simulink model "solar_tracker"  (R2026b)
settings: Solver=ode4  StopTime=cfg.simulation.durationHours * 3600  FixedStep=cfg.simulation.energySampleTime
model workspace (MAT data in the model file):
  targetAzimuthInput = timeseries
  targetAzimuthInput.Name = 'unnamed'
  targetAzimuthInput.DataInfo = tsdata.datametadata
  targetAzimuthInput.DataInfo.Interpolation = tsdata.interpolation
  targetAzimuthInput.DataInfo.Interpolation.Fhandle : function handle (value not decoded)
  targetAzimuthInput.DataInfo.Interpolation.Name = 'linear'
  targetAzimuthInput.TimeInfo = tsdata.timemetadata
  targetAzimuthInput.TimeInfo.Length = 2
  targetAzimuthInput.TimeInfo.DuplicateTimes = 0
  targetAzimuthInput.TimeInfo.Time_ = [0; 86400]
  targetAzimuthInput.TimeInfo.Initialized = 1
  targetAzimuthInput.QualityInfo = tsdata.qualmetadata
  targetAzimuthInput.Data_ = [0; 0]
  targetTiltInput = timeseries
  targetTiltInput.Name = 'unnamed'
  targetTiltInput.DataInfo = tsdata.datametadata
  targetTiltInput.DataInfo.Interpolation = tsdata.interpolation
  targetTiltInput.DataInfo.Interpolation.Fhandle : function handle (value not decoded)
  targetTiltInput.DataInfo.Interpolation.Name = 'linear'
  targetTiltInput.TimeInfo = tsdata.timemetadata
  targetTiltInput.TimeInfo.Length = 2
  targetTiltInput.TimeInfo.DuplicateTimes = 0
  targetTiltInput.TimeInfo.Time_ = [0; 86400]
  targetTiltInput.TimeInfo.Initialized = 1
  targetTiltInput.QualityInfo = tsdata.qualmetadata
  targetTiltInput.Data_ = [0; 0]
values from neighbouring files (symbols this model uses):
  cfg = project_config()    [validate_tracker_plant.m]    (also in verify_axis_plant.m)
settings Model: Creator=Jhons Janner Samuel  LastModifiedBy=Jhons Janner Samuel

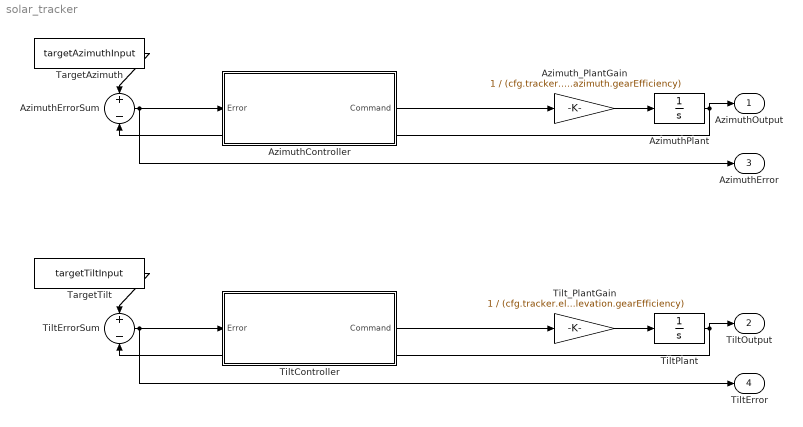
== system solar_tracker ==
  AzimuthController : Subsystem
  AzimuthErrorSum : Sum  Inputs=+-
  AzimuthPlant : Integrator
  Azimuth_PlantGain : Gain  Gain=1 / (cfg.tracker.azimuth.gearRatio * cfg.tracker.azimuth.gearEfficiency)
  TargetAzimuth : FromWorkspace  VariableName=targetAzimuthInput
  TargetTilt : FromWorkspace  VariableName=targetTiltInput
  TiltController : Subsystem
  TiltErrorSum : Sum  Inputs=+-
  TiltPlant : Integrator
  Tilt_PlantGain : Gain  Gain=1 / (cfg.tracker.elevation.gearRatio * cfg.tracker.elevation.gearEfficiency)
  AzimuthOutput : Outport
  TiltOutput : Outport  Port=2
  AzimuthError : Outport  Port=3
  TiltError : Outport  Port=4
  wires:
  TargetAzimuth/1 -> AzimuthErrorSum/1
  TargetTilt/1 -> TiltErrorSum/1
  AzimuthErrorSum/1 -> AzimuthController/1(Error), AzimuthError/1
  AzimuthController/1(Command) -> Azimuth_PlantGain/1
  Azimuth_PlantGain/1 -> AzimuthPlant/1
  AzimuthPlant/1 -> AzimuthOutput/1, AzimuthErrorSum/2
  TiltErrorSum/1 -> TiltController/1(Error), TiltError/1
  TiltController/1(Command) -> Tilt_PlantGain/1
  Tilt_PlantGain/1 -> TiltPlant/1
  TiltPlant/1 -> TiltOutput/1, TiltErrorSum/2

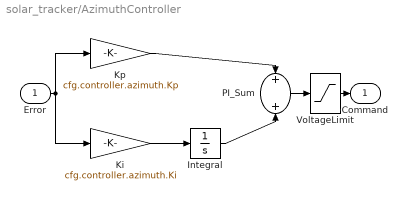
== system solar_tracker/AzimuthController ==
  Error : Inport
  Integral : Integrator
  Ki : Gain  Gain=cfg.controller.azimuth.Ki
  Kp : Gain  Gain=cfg.controller.azimuth.Kp
  PI_Sum : Sum
  VoltageLimit : Saturate  UpperLimit=cfg.controller.azimuth.outputMax  LowerLimit=cfg.controller.azimuth.outputMin
  Command : Outport
  wires:
  Error/1 -> Kp/1, Ki/1
  Ki/1 -> Integral/1
  Kp/1 -> PI_Sum/1
  Integral/1 -> PI_Sum/2
  PI_Sum/1 -> VoltageLimit/1
  VoltageLimit/1 -> Command/1

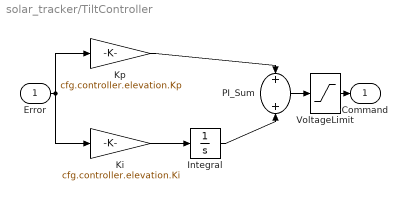
== system solar_tracker/TiltController ==
  Error : Inport
  Integral : Integrator
  Ki : Gain  Gain=cfg.controller.elevation.Ki
  Kp : Gain  Gain=cfg.controller.elevation.Kp
  PI_Sum : Sum
  VoltageLimit : Saturate  UpperLimit=cfg.controller.elevation.outputMax  LowerLimit=cfg.controller.elevation.outputMin
  Command : Outport
  wires:
  Error/1 -> Kp/1, Ki/1
  Ki/1 -> Integral/1
  Kp/1 -> PI_Sum/1
  Integral/1 -> PI_Sum/2
  PI_Sum/1 -> VoltageLimit/1
  VoltageLimit/1 -> Command/1
